simulink model "arduino_pil"  (R2023a)
settings: Solver=FixedStepDiscrete  StartTime=0.0  StopTime=10  RelTol=1e-3
PostLoadFcn:
  | Increment = Simulink.Parameter;
  | Increment.DataType = 'uint8';
  | Increment.CoderInfo.StorageClass = 'SimulinkGlobal';
  | Increment.Value = 1;
  | 
  | SilCounterBus = Simulink.Bus;
  | SilCounterBus.Description = 'This bus contains counter inputs';
  | 
  | e1 = Simulink.BusElement;
  | e1.DataType = 'boolean';
  | e1.Name = 'ticks_to_count';
  | 
  | e2 = Simulink.BusElement;
  | e2.DataType = 'boolean';
  | e2.Name = 'reset';
  | 
  | SilCounterBus.Elements = [e1 e2];
  | clear e1 e2
  | 
  | % Step size
  | T=0.1;
  | 
  | % Input values
  | ticks_to_count.time = (0:100)'*T;
  | ticks_to_count.signals.values = boolean((floor( (0:100)/2)==(0:100)/2)');
  | ticks_to_count.signals.dimensions = 1;
  | 
  | reset.time = (0:100)'*T;
  | reset_values = boolean(zeros(101,1)); reset_values(20)=true;
  | reset.signals.values = reset_values;
  | clear reset_values
  | reset.signals.dimensions = 1;
model workspace (MATLAB code in the model file):
  | myLower = Simulink.Parameter;
  | myLower.Value = uint8(20);
  | 
  | myUpper = Simulink.Parameter;
  | myUpper.Value = uint8(40);
libraries: arduinolib x4, arduinosensorlib x1
Description:
  | Example model reference component.
settings Model: ModifiedByFormat=The MathWorks Inc.  ExtModeTrigDuration=2  Creator=The MathWorks, Inc.  LastModifiedBy=The MathWorks Inc.
settings SolverCC: AlgebraicLoopSolver=TrustRegion  PositivePriorityOrder=on
settings DataIOCC: SaveFormat=StructureWithTime  SaveOutput=off  SaveTime=off  ReturnWorkspaceOutputs=off  SignalLoggingName=logsOut
settings OptimizationCC: UseDivisionForNetSlopeComputation=UseDivisionForReciprocalsOfIntegersOnly  DefaultUnderspecifiedDataType=single  EnhancedBackFolding=on  BooleansAsBitfields=on  PassReuseOutputArgsAs=Individual arguments  ExpressionDepthLimit=2147483647  StateBitsets=on  DataBitsets=on  ZeroExternalMemoryAtStartup=off  ZeroInternalMemoryAtStartup=off  NoFixptDivByZeroProtection=on  EfficientFloat2IntCast=on  LifeSpan=1  MaxStackSize=64  SimCompilerOptimization=on  EfficientTunableParamExpr=on
settings DebuggingCC: ReadBeforeWriteMsg=DisableAll  WriteAfterWriteMsg=DisableAll  WriteAfterReadMsg=DisableAll  UnderspecifiedInitializationDetection=Classic  CheckExecutionContextPreStartOutputMsg=on  ParameterPrecisionLossMsg=none  FcnCallInpInsideContextMsg=warning  UnconnectedInputMsg=warning  UnconnectedOutputMsg=warning  UnconnectedLineMsg=warning  UniqueDataStoreMsg=error  AllowSymbolicDim=off  ModelReferenceSymbolNameMessage=none  StateNameClashWarn=warning  StrictBusMsg=ErrorOnBusTreatedAsVector  SFUnexpectedBacktrackingDiag=warning  SFNoUnconditionalDefaultTransitionDiag=warning  SFExecutionAtInitializationDiag=none  ArithmeticOperatorsInVariantConditions=warning
settings HardwareCC: ProdBitPerInt=16  ProdBitPerPointer=16  ProdBitPerSizeT=16  ProdBitPerPtrDiffT=16  ProdLargestAtomicFloat=None  ProdWordSize=8  ProdHWDeviceType=Atmel->AVR  TargetHWDeviceType=Generic->32-bit Embedded Processor
settings ModelReferenceCC: EnableRefExpFcnMdlSchedulingChecks=on  CheckModelReferenceTargetMessage=none  PropagateVarSize=During execution  ModelReferencePassRootInputsByReference=off  PropagateSignalLabelsOutOfModel=off
settings SFSimCC: SimUseLocalCustomCode=off  MATLABDynamicMemAlloc=off
settings RTWCC: Description=Embedded Coder  SystemTargetFile=ert.tlc  HardwareBoard=Arduino Mega 2560  TemplateMakefile=ert_default_tmf  GenerateReport=on  RTWVerbose=off  RTWUseLocalCustomCode=off  Toolchain=Arduino AVR  BuildConfiguration=Faster Runs  IncludeHyperlinkInReport=on  PortableWordSizes=on  GenerateTraceInfo=on  GenerateTraceReport=on  GenerateTraceReportSl=on  GenerateTraceReportSf=on  GenerateTraceReportEml=on  DLArmComputeVersion=19.05
settings CodeAppCC: ForceParamTrailComments=on  IgnoreCustomStorageClasses=off  SimulinkDataObjDesc=on  CustomSymbolStrGlobalVar=rt$N$M  CustomSymbolStrType=$N$M  CustomSymbolStrFcn=$N$M$F  CustomSymbolStrModelFcn=$N  CustomSymbolStrMacro=$N$M  InsertBlockDesc=on  StateflowObjectComments=on  InternalIdentifier=Classic
settings ERTTargetCC: UtilityFuncGeneration=Shared location  MultiwordLength=2048  IncludeMdlTerminateFcn=off  CombineSignalStateStructs=on  SupportAbsoluteTime=off  SupportNonFinite=off  SupportComplex=off  SupportVariableSizeSignals=on  ERTFilePackagingFormat=CompactWithDataFile  ConvertIfToSwitch=off  SuppressUnreachableDefaultCases=off
settings ConfigComp: CovMetricSettings=dw  CovSaveCumulativeToWorkspaceVar=on  CovSaveSingleToWorkspaceVar=on  CovExternalEMLEnable=off  CovSFcnEnable=off

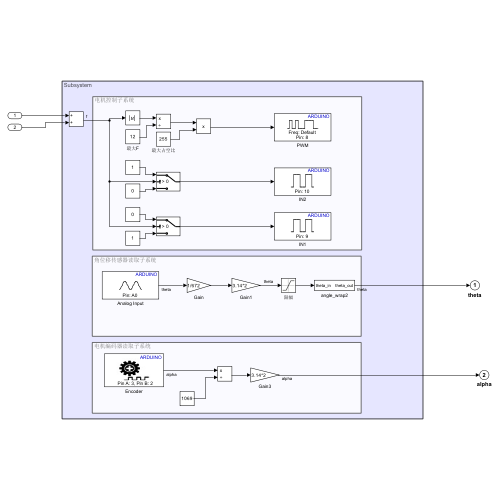
[thumbnail: Simulink's stored preview of the top-level diagram]
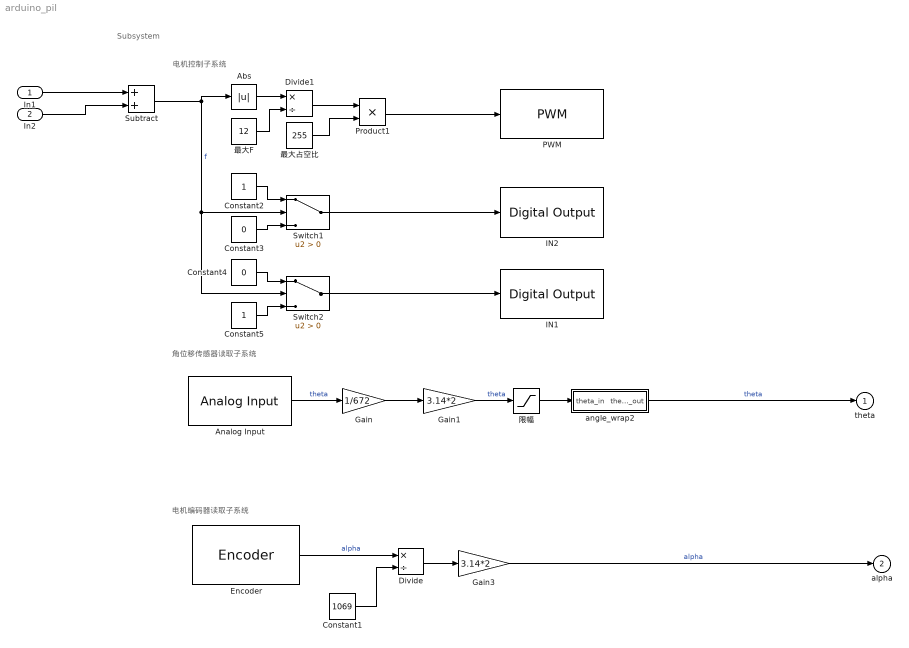
== system arduino_pil ==
  note: Subsystem
  note: 电机控制子系统
  note: 角位移传感器读取子系统
  note: 电机编码器读取子系统
  In1 : Inport
  In2 : Inport  Port=2
  Abs : Abs  OutDataTypeStr=single  SaturateOnIntegerOverflow=off
  Analog Input : arduinolib/Analog Input  pinNumber=0  ReadResultsOnly=off  ConversionTriggerSource=Software  ExternalTriggerType=uint32( 0 )  OutputDataType=uint16  EnableConversionCompleteNotify=off  EnableOuputStatus=off  SampleTime=-1  blockPlatform=arduino
  Constant1 : Constant  Value=1069  OutDataTypeStr=single
  Constant2 : Constant  OutDataTypeStr=single
  Constant3 : Constant  Value=0  OutDataTypeStr=single
  Constant4 : Constant  Value=0  OutDataTypeStr=single
  Constant5 : Constant  OutDataTypeStr=single
  Divide : Product  Inputs=*/  OutDataTypeStr=single
  Divide1 : Product  Inputs=*/  OutDataTypeStr=single
  Encoder : arduinosensorlib/Encoder  InputA=3  InputB=2  Mode=No reset  SampleTime=-1
  Gain : Gain  Gain=1/672  OutDataTypeStr=single
  Gain1 : Gain  Gain=3.14*2  OutDataTypeStr=single
  Gain3 : Gain  Gain=3.14*2  OutDataTypeStr=single
  IN1 : arduinolib/Digital Output  pinNumber=9  Direction=output  blockPlatform=arduino
  IN2 : arduinolib/Digital Output  pinNumber=10  Direction=output  blockPlatform=arduino
  PWM : arduinolib/PWM  pinNumber=8  frequencyType=Default  desiredFrequency=490.2  achievableFrequency=490.2
  Product1 : Product  OutDataTypeStr=single
  Subtract : Sum  OutDataTypeStr=single
  Switch1 : Switch  Criteria=u2 > Threshold  OutDataTypeStr=single  SaturateOnIntegerOverflow=off  InputSameDT=off
  Switch2 : Switch  Criteria=u2 > Threshold  OutDataTypeStr=single  SaturateOnIntegerOverflow=off  InputSameDT=off
  angle_wrap2 : Subsystem
  最大F : Constant  Value=12  OutDataTypeStr=single
  最大占空比 : Constant  Value=255  OutDataTypeStr=single
  限幅 : Saturate  UpperLimit=6.28  LowerLimit=0  OutDataTypeStr=single
  theta : Outport  OutDataTypeStr=single  VectorParamsAs1DForOutWhenUnconnected=off
  alpha : Outport  Port=2  OutDataTypeStr=single  VectorParamsAs1DForOutWhenUnconnected=off
  wires:
  Constant2/1 -> Switch1/1
  Analog Input/1 -> Gain/1  "theta"
  Switch1/1 -> IN2/1
  Product1/1 -> PWM/1
  Constant4/1 -> Switch2/1
  Abs/1 -> Divide1/1
  最大F/1 -> Divide1/2
  Gain/1 -> Gain1/1
  Constant5/1 -> Switch2/3
  最大占空比/1 -> Product1/2
  Divide/1 -> Gain3/1
  Switch2/1 -> IN1/1
  Subtract/1 -> Switch2/2, Switch1/2, Abs/1  "f"
  限幅/1 -> angle_wrap2/1(theta_in)
  Gain1/1 -> 限幅/1  "theta"
  Constant3/1 -> Switch1/3
  Constant1/1 -> Divide/2
  Divide1/1 -> Product1/1
  Gain3/1 -> alpha/1  "alpha"
  Encoder/1 -> Divide/1  "alpha"
  In1/1 -> Subtract/1
  In2/1 -> Subtract/2
  angle_wrap2/1(theta_out) -> theta/1  "theta"

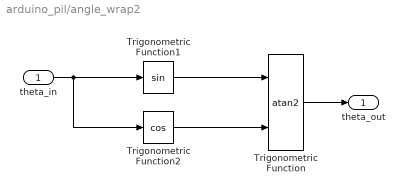
== system arduino_pil/angle_wrap2 ==
  theta_in : Inport
  Trigonometric Function : Trigonometry  Operator=atan2
  Trigonometric Function1 : Trigonometry
  Trigonometric Function2 : Trigonometry  Operator=cos
  theta_out : Outport  VectorParamsAs1DForOutWhenUnconnected=off
  wires:
  Trigonometric Function2/1 -> Trigonometric Function/2
  Trigonometric Function1/1 -> Trigonometric Function/1
  Trigonometric Function/1 -> theta_out/1
  theta_in/1 -> Trigonometric Function1/1, Trigonometric Function2/1
